simulink model "turtlebot_odomtest"  (R2026a)
settings: Solver=FixedStepAuto  StopTime=inf  FixedStep=0.1
undefined symbols (not defined in the file): Angular, Linear
libraries: robotlib x3
settings Model: Creator=linuxpc  LastModifiedBy=linuxpc

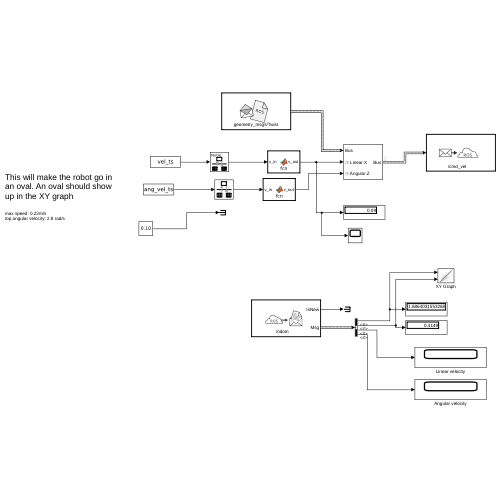
[thumbnail: Simulink's stored preview of the top-level diagram]
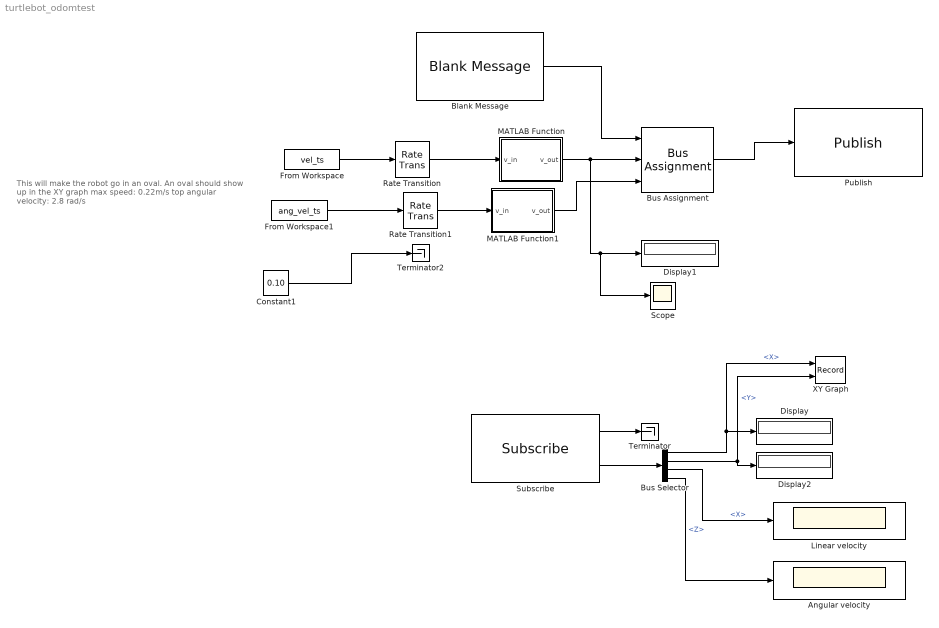
== system turtlebot_odomtest ==
  note: This will make the robot go in an oval. An oval should show up in the XY graph
      |
      | max speed: 0.22m/s
      | top angular velocity: 2.8 rad/s
  Angular velocity : Scope
      settings: ActiveDisplayYMinimum=-0.0776605389634265  ActiveDisplayYMaximum=0.055433328139946725
  Blank Message : robotlib/Blank Message  messageClass=Message  entityType=geometry_msgs/Twist  messageType=geometry_msgs/Twist  SampleTime=0.1  legacyBusStruct=off
  Bus Assignment : BusAssignment  AssignedSignals=Linear.X,Angular.Z
  Bus Selector : BusSelector  OutputSignals=Pose.Pose.Position.X,Pose.Pose.Position.Y,Twist.Twist.Linear.X,Twist.Twist.Angular.Z
  Constant1 : Constant  Value=0.10
  Display : Display
      settings: Format=decimal (Stored Integer)
  Display1 : Display
  Display2 : Display
  From Workspace : FromWorkspace  VariableName=vel_ts  SampleTime=0.1  Interpolate=off  OutputAfterFinalValue=Holding final value
  From Workspace1 : FromWorkspace  VariableName=ang_vel_ts  SampleTime=0.1  Interpolate=off  OutputAfterFinalValue=Holding final value
  Linear velocity : Scope
      settings: ActiveDisplayYMinimum=-0.80895325167692544  ActiveDisplayYMaximum=0.758099081259992
  MATLAB Function : MATLAB Function  TreatAsAtomicUnit=on
  MATLAB Function1 : MATLAB Function  TreatAsAtomicUnit=on
  Publish : robotlib/Publish  topicSource=Select from ROS network  topic=/cmd_vel  messageType=geometry_msgs/Twist  legacyBusStruct=off  messageQueueLength=1
  Rate Transition : RateTransition  OutPortSampleTime=0.1
  Rate Transition1 : RateTransition  OutPortSampleTime=0.1
  Scope : Scope
      settings: ActiveDisplayYMinimum=-0.31933816600271908  ActiveDisplayYMaximum=0.27765381765477576  DataLoggingVariableName=ScopeData2
  Subscribe : robotlib/Subscribe  topicSource=Select from ROS network  topic=/odom  messageType=nav_msgs/Odometry  SampleTime=-1  legacyBusStruct=off  messageQueueLength=1
  Terminator : Terminator
  Terminator2 : Terminator
  XY Graph : Record  NumPorts=2.0  FileSettingsInternal="{\"entries\":[{\"content\":{\"excelSettings\":{\"content\":{},\"type\":\"Streamout.ExcelSettings\"},\"parquetSettings\":{\"content\":{},\"type\":\"Streamout.ParquetSettings\"}},\"type\":\"Streamout.FileSettingStorage\",\"uuid\":\"\"}],\"packageUris\":[\"http:\\/\\/schema.mathworks.com\\/mf0\\/streamout_blocks\\/R2020a\"],\"version\":\"1.0\"}"  FrameSettings=[0, 0]  Layout=[1 1]  SignalsInternal="{\"entries\":[{\"content\":{\"signals\":[{\"content\":{\"blockPath\":[],\"dimensions\":[1],\"domain\":\"\",\"lineColor\":\"#a2142f\",\"plots\":[ 1 ],\"port\":1,\"sid\":[\"\"],\"signalID\":1,\"signalName\":\"<X>\"},\"type\":\"RecordBlkView.Signal\",\"uuid\":\"\"},{\"content\":{\"blockPath\":[],\"dimensions\":[1],\"domain\":\"\",\"lineColor\":\"#139fff\",\"plots\":[ 1 ],\"port\":2,\"sid\":[\"\"],\"signalID\":2,\"signalName\":\"<Y>\"},\"type\":\"RecordBlkView.Signal\",\"uuid\":\"\"}]},\"type\":\"RecordBlkView.InputSignals\",\"uuid\":\"\"}],\"packageUris\":[\"http:\\/\\/schema.mathworks.com\\/mf0\\/streamout_blocks\\/R2020a\"],\"version\":\"1.0\"}"  VisualizationBindings="{\"xyplotplugin\":{\"info\":[{\"series\":[{\"bindingParametersList\":[{\"parameter\":\"X-Axis\",\"signalID\":1,\"signalName\":\"<X>\"},{\"parameter\":\"Y-Axis\",\"signalID\":2,\"signalName\":\"<Y>\"}],\"seriesID\":0}],\"subplotID\":1}]}}"  CompatibilityTag=XY
  wires:
  Subscribe/2 -> Bus Selector/1
  Bus Selector/1 -> XY Graph/1, Display/1  "<X>"
  Subscribe/1 -> Terminator/1
  Blank Message/1 -> Bus Assignment/1
  Bus Assignment/1 -> Publish/1
  Bus Selector/2 -> Display2/1, XY Graph/2  "<Y>"
  MATLAB Function/1(v_out) -> Scope/1, Display1/1, Bus Assignment/2
  Bus Selector/3 -> Linear velocity/1  "<X>"
  Bus Selector/4 -> Angular velocity/1  "<Z>"
  Constant1/1 -> Terminator2/1
  MATLAB Function1/1(v_out) -> Bus Assignment/3
  From Workspace/1 -> Rate Transition/1
  From Workspace1/1 -> Rate Transition1/1
  Rate Transition/1 -> MATLAB Function/1(v_in)
  Rate Transition1/1 -> MATLAB Function1/1(v_in)

== matlab function turtlebot_odomtest/MATLAB Function ==
  data: v_in input; v_out output
function v_out = fcn(v_in)
    if v_in == 0
        v_out = 0.01;   % tiny creep instead of full stop
    else
        v_out = v_in;
    end
end

== matlab function turtlebot_odomtest/MATLAB Function1 ==
  data: v_in input; v_out output
function v_out = fcn(v_in)
    if v_in == 0
        v_out = 0;   % tiny creep instead of full stop
    else
        v_out = v_in;
    end
end
